simulink model "sanxiangnibianqiaoshidianyaxing"  (R2025a)
settings: Solver=ode23tb  StartTime=0.0  StopTime=0.2  MaxStep=1e-5  RelTol=1e-5
libraries: spsIGBTDiodeLib x6, spsThreePhaseSeriesRLCBranchLib x6, spsDCVoltageSourceLib x2, spsVoltageMeasurementLib x2, spsUniversalBridgeLib x1, sps_lib x1
settings Model: Creator=hdl  LastModifiedBy=hdl

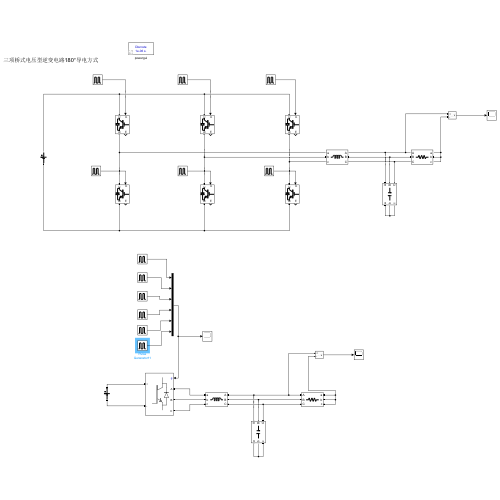
[thumbnail: Simulink's stored preview of the top-level diagram]
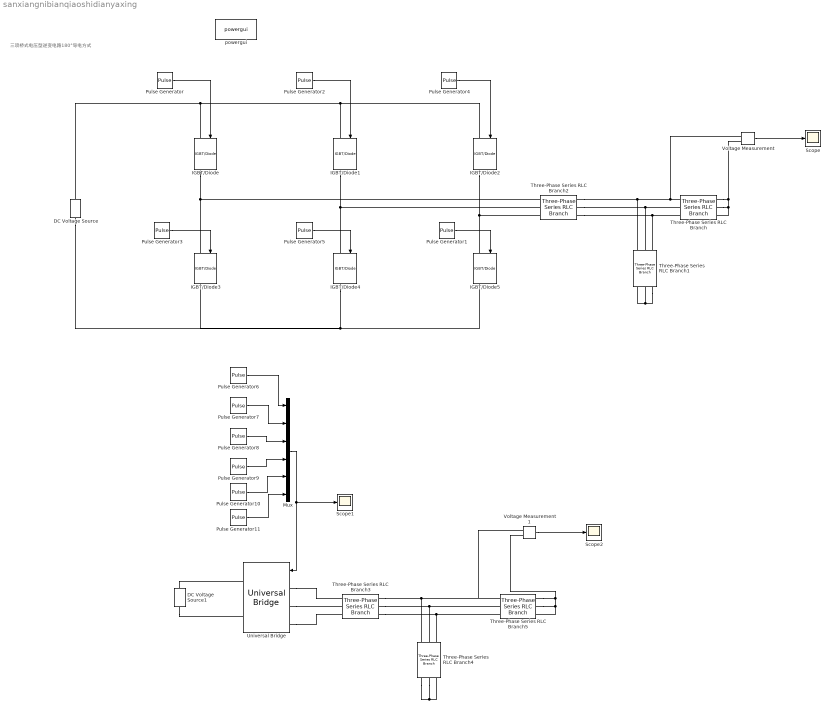
== system sanxiangnibianqiaoshidianyaxing ==
  note: 三项桥式电压型逆变电路180°导电方式
  DC Voltage Source : spsDCVoltageSourceLib/DC Voltage Source  Amplitude=100  Measurements=None
  DC Voltage Source1 : spsDCVoltageSourceLib/DC Voltage Source  Amplitude=100  Measurements=None
  IGBT/Diode{,1..5} (6 alike) : spsIGBTDiodeLib/IGBT//Diode  Ron=1e-3  Rs=1e5  Cs=inf  Measurements=on
  Mux : Mux  Inputs=6
  Pulse Generator : DiscretePulseGenerator  PulseType=Time based  Period=1/1e4  PulseWidth=50
  Pulse Generator1 : DiscretePulseGenerator  PulseType=Time based  Period=1/1e4  PulseWidth=50  PhaseDelay=1/1e4*1/6
  Pulse Generator10 : DiscretePulseGenerator  PulseType=Time based  Period=1/1e4  PulseWidth=50  PhaseDelay=1/1e4*4/6
  Pulse Generator11 : DiscretePulseGenerator  PulseType=Time based  Period=1/1e4  PulseWidth=50  PhaseDelay=1/1e4*1/6
  Pulse Generator2 : DiscretePulseGenerator  PulseType=Time based  Period=1/1e4  PulseWidth=50  PhaseDelay=1/1e4*2/6
  Pulse Generator3 : DiscretePulseGenerator  PulseType=Time based  Period=1/1e4  PulseWidth=50  PhaseDelay=1/1e4*3/6
  Pulse Generator4 : DiscretePulseGenerator  PulseType=Time based  Period=1/1e4  PulseWidth=50  PhaseDelay=1/1e4*4/6
  Pulse Generator5 : DiscretePulseGenerator  PulseType=Time based  Period=1/1e4  PulseWidth=50  PhaseDelay=1/1e4*5/6
  Pulse Generator6 : DiscretePulseGenerator  PulseType=Time based  Period=1/1e4  PulseWidth=50
  Pulse Generator7 : DiscretePulseGenerator  PulseType=Time based  Period=1/1e4  PulseWidth=50  PhaseDelay=1/1e4*3/6
  Pulse Generator8 : DiscretePulseGenerator  PulseType=Time based  Period=1/1e4  PulseWidth=50  PhaseDelay=1/1e4*2/6
  Pulse Generator9 : DiscretePulseGenerator  PulseType=Time based  Period=1/1e4  PulseWidth=50  PhaseDelay=1/1e4*5/6
  Scope : Scope
      settings: ActiveDisplayYMinimum=-92.54064386372832  ActiveDisplayYMaximum=92.54064397079992
  Scope1 : Scope
      settings: ActiveDisplayYMinimum=-1.239216739248771  ActiveDisplayYMaximum=1.6216942272217592
  Scope2 : Scope
      settings: ActiveDisplayYMinimum=-92.54064386372832  ActiveDisplayYMaximum=92.54064397079992  DataLoggingVariableName=ScopeData2
  Three-Phase Series RLC Branch : spsThreePhaseSeriesRLCBranchLib/Three-Phase Series RLC Branch  LConnTagsString=A|B|C  RConnTagsString=A|B|C  BranchType=R  Resistance=1  Inductance=1e-3  Capacitance=1e-6  Measurements=None
  Three-Phase Series RLC Branch1 : spsThreePhaseSeriesRLCBranchLib/Three-Phase Series RLC Branch  LConnTagsString=A|B|C  RConnTagsString=A|B|C  BranchType=C  Resistance=1  Inductance=1e-3  Capacitance=1e-5  Measurements=None
  Three-Phase Series RLC Branch2 : spsThreePhaseSeriesRLCBranchLib/Three-Phase Series RLC Branch  LConnTagsString=A|B|C  RConnTagsString=A|B|C  BranchType=L  Resistance=1  Inductance=1e-5  Capacitance=1e-2  Measurements=None
  Three-Phase Series RLC Branch3 : spsThreePhaseSeriesRLCBranchLib/Three-Phase Series RLC Branch  LConnTagsString=A|B|C  RConnTagsString=A|B|C  BranchType=L  Resistance=1  Inductance=1e-5  Capacitance=1e-2  Measurements=None
  Three-Phase Series RLC Branch4 : spsThreePhaseSeriesRLCBranchLib/Three-Phase Series RLC Branch  LConnTagsString=A|B|C  RConnTagsString=A|B|C  BranchType=C  Resistance=1  Inductance=1e-3  Capacitance=1e-5  Measurements=None
  Three-Phase Series RLC Branch5 : spsThreePhaseSeriesRLCBranchLib/Three-Phase Series RLC Branch  LConnTagsString=A|B|C  RConnTagsString=A|B|C  BranchType=R  Resistance=1  Inductance=1e-3  Capacitance=1e-6  Measurements=None
  Universal Bridge : spsUniversalBridgeLib/Universal Bridge  Arms=3  SnubberResistance=1e5  SnubberCapacitance=inf  Device=IGBT / Diodes  Ron=1e-3  Lon=0  ForwardVoltages="[  0  0  ]"  ForwardVoltage=0  GTOparameters=[ 10e-6 , 20e-6 ]  IGBTparameters=[ 1e-6 , 2e-6 ]  Measurements=None  Measurements_2=None  converterType=Rectifier
  Voltage Measurement : spsVoltageMeasurementLib/Voltage Measurement  PhasorSimulation=off  OutputType=Complex  PSBequivalent=0
  Voltage Measurement1 : spsVoltageMeasurementLib/Voltage Measurement  PhasorSimulation=off  OutputType=Complex  PSBequivalent=0
  powergui : sps_lib/powergui  Priority=1  SimulationMode=Discrete  SampleTime=1e-6  frequency=60  Iterations=50  frequencyindice=0  Pbase=100e6  ErrMax=1e-4  UnitsV=kV  UnitsW=MW  buscounter=0  FunctionMessages=off  echomessages=off  EnableUseOfTLC=off  CurrentSourceSwitches=off  DisableSnubberDevices=off  DisableRonSwitches=off  DisableVfSwitches=off  DisplayEquations=off  AutomaticDiscreteSolvers=off  SolverType=Tustin/Backward Euler (TBE)  Interpol=off  ExternalGateDelay=off  methode=off  Ts=100  x0status=blocks  SPID=on  SwTol=0  HookPort=off  NonlinearTolerance=1e-4  nMaxIteration=100  ContinueOnMaxIteration=off  RestoreLinks=warning  ResistiveCurrentMeasurement=off  Frange=[0:2:500]  Ylog=off  Xlog=on  ShowGrid=off  save=off  variable=ZData  structure=0  ZoomFFT=off  StartTime=0.0  cycles=1  DisplayStyle=1  fundamental=60  FreqAxis=off  MaxFrequency=1000  frequencyindicesteady=1  RmsSteady=1  display=off
  wires:
  Pulse Generator/1 -> IGBT/Diode/1
  Pulse Generator3/1 -> IGBT/Diode3/1
  Pulse Generator2/1 -> IGBT/Diode1/1
  Pulse Generator4/1 -> IGBT/Diode2/1
  Pulse Generator5/1 -> IGBT/Diode4/1
  Pulse Generator1/1 -> IGBT/Diode5/1
  Voltage Measurement/1 -> Scope/1
  Pulse Generator7/1 -> Mux/2
  Pulse Generator6/1 -> Mux/1
  Pulse Generator8/1 -> Mux/3
  Pulse Generator9/1 -> Mux/4
  Pulse Generator10/1 -> Mux/5
  Pulse Generator11/1 -> Mux/6
  Mux/1 -> Scope1/1, Universal Bridge/1
  Voltage Measurement1/1 -> Scope2/1
  connections:
  DC Voltage Source/LConn1 -- IGBT/Diode3/RConn1 -- IGBT/Diode4/RConn1 -- IGBT/Diode5/RConn1
  DC Voltage Source/RConn1 -- IGBT/Diode/LConn1 -- IGBT/Diode2/LConn1 -- IGBT/Diode1/LConn1
  Three-Phase Series RLC Branch/LConn1 -- Three-Phase Series RLC Branch2/LConn1 -- Three-Phase Series RLC Branch1/LConn1 -- Voltage Measurement/LConn1
  IGBT/Diode1/RConn1 -- Three-Phase Series RLC Branch2/RConn2 -- IGBT/Diode4/LConn1
  Three-Phase Series RLC Branch1/LConn3 -- Three-Phase Series RLC Branch2/LConn3 -- Three-Phase Series RLC Branch/LConn3
  Three-Phase Series RLC Branch/RConn1 -- Voltage Measurement/LConn2 -- Three-Phase Series RLC Branch/RConn2 -- Three-Phase Series RLC Branch/RConn3
  Three-Phase Series RLC Branch1/RConn3 -- Three-Phase Series RLC Branch1/RConn1 -- Three-Phase Series RLC Branch1/RConn2
  IGBT/Diode/RConn1 -- Three-Phase Series RLC Branch2/RConn1 -- IGBT/Diode3/LConn1
  Three-Phase Series RLC Branch/LConn2 -- Three-Phase Series RLC Branch2/LConn2 -- Three-Phase Series RLC Branch1/LConn2
  IGBT/Diode2/RConn1 -- Three-Phase Series RLC Branch2/RConn3 -- IGBT/Diode5/LConn1
  DC Voltage Source1/RConn1 -- Universal Bridge/RConn1
  DC Voltage Source1/LConn1 -- Universal Bridge/RConn2
  Universal Bridge/LConn2 -- Three-Phase Series RLC Branch3/RConn2
  Universal Bridge/LConn1 -- Three-Phase Series RLC Branch3/RConn1
  Universal Bridge/LConn3 -- Three-Phase Series RLC Branch3/RConn3
  Three-Phase Series RLC Branch3/LConn3 -- Three-Phase Series RLC Branch5/LConn3 -- Three-Phase Series RLC Branch4/LConn3
  Three-Phase Series RLC Branch3/LConn2 -- Three-Phase Series RLC Branch5/LConn2 -- Three-Phase Series RLC Branch4/LConn2
  Three-Phase Series RLC Branch3/LConn1 -- Voltage Measurement1/LConn1 -- Three-Phase Series RLC Branch5/LConn1 -- Three-Phase Series RLC Branch4/LConn1
  Three-Phase Series RLC Branch5/RConn1 -- Voltage Measurement1/LConn2 -- Three-Phase Series RLC Branch5/RConn2 -- Three-Phase Series RLC Branch5/RConn3
  Three-Phase Series RLC Branch4/RConn1 -- Three-Phase Series RLC Branch4/RConn2 -- Three-Phase Series RLC Branch4/RConn3
